simulink model "H175_V3_walk"  (R2025b)
(part 3 of 13)

  L_little1/LConn1 -- L_wrist_yaw1/RConn4
  L_middle1/LConn1 -- L_wrist_yaw1/RConn3
  L_elbow/RConn1 -- L_elbow1/LConn1
  L_ring1/LConn1 -- L_wrist_yaw1/RConn2
  L_thumb1/LConn1 -- L_wrist_yaw1/RConn1
  R_ankle_pitch/RConn1 -- R_ankle_pitch1/LConn1
  R_ankle_pitch1/RConn1 -- R_ankle_roll/LConn1
  R_ankle_roll/RConn1 -- ct_rot_R1/LConn1 -- ct_rot_R2/LConn1 -- ct_rot_R3/LConn1 -- R_ankle_roll1/LConn1 -- ct_rot_R4/LConn1
  R_ankle_roll1/RConn1 -- R_toe/LConn1
  R_clavicle/RConn1 -- R_clavicle1/LConn1
  R_clavicle1/RConn1 -- R_shoulder_pitch/LConn1
  R_elbow/RConn1 -- R_elbow1/LConn1
  R_elbow1/RConn1 -- R_forearm_twist/LConn1
  L_elbow1/RConn1 -- L_forearm_twist/LConn1
  R_forearm_twist/RConn1 -- R_forearm_twist1/LConn1
  R_forearm_twist1/RConn1 -- R_wrist_pitch/LConn1
  R_hip_pitch/RConn1 -- R_hip_pitch1/LConn1
  R_hip_pitch1/RConn1 -- R_hip_roll/LConn1
  R_hip_roll/RConn1 -- R_hip_roll1/LConn1
  R_hip_roll1/RConn1 -- R_hip_yaw/LConn1
  R_hip_yaw/RConn1 -- R_hip_yaw1/LConn1
  R_hip_yaw1/RConn1 -- R_knee/LConn1
  R_index1/RConn1 -- R_index4/LConn1
  R_index2/LConn1 -- R_index4/RConn1
  L_forearm_twist/RConn1 -- L_forearm_twist1/LConn1
  R_index2/RConn1 -- R_index5/LConn1
  R_index3/LConn1 -- R_index5/RConn1
  R_index3/RConn1 -- R_index6/LConn1
  R_knee/RConn1 -- R_knee1/LConn1
  R_ankle_pitch/LConn1 -- R_knee1/RConn1
  R_little1/RConn1 -- R_little4/LConn1
  R_little2/LConn1 -- R_little4/RConn1
  R_little2/RConn1 -- R_little5/LConn1
  R_little3/LConn1 -- R_little5/RConn1
  R_little3/RConn1 -- R_little6/LConn1
  L_forearm_twist1/RConn1 -- L_wrist_pitch/LConn1
  R_middle1/RConn1 -- R_middle4/LConn1
  R_middle2/LConn1 -- R_middle4/RConn1
  R_middle2/RConn1 -- R_middle5/LConn1
  R_middle3/LConn1 -- R_middle5/RConn1
  R_middle3/RConn1 -- R_middle6/LConn1
  R_ring1/RConn1 -- R_ring4/LConn1
  R_ring2/LConn1 -- R_ring4/RConn1
  R_ring2/RConn1 -- R_ring5/LConn1
  R_ring3/LConn1 -- R_ring5/RConn1
  R_ring3/RConn1 -- R_ring6/LConn1
  Solver Configuration/RConn1 -- MechanismConfiguration/RConn1 -- FloatingBase/LConn1 -- GroundTf/LConn1 -- ps_X/LConn1 -- ps_Y/LConn1 -- ps_XDot/LConn1 -- World/RConn1 -- ps_YDot/LConn1
  FloatingBase/RConn1 -- ps_X/RConn1 -- ps_Y/RConn1 -- ps_XDot/RConn1 -- pelvis/LConn1 -- ps_YDot/RConn1
  Ground/RConn1 -- GroundTf/RConn1 -- gnd_L1/RConn1 -- gnd_L2/RConn1 -- gnd_L3/RConn1 -- gnd_L4/RConn1 -- gnd_R1/RConn1 -- gnd_R2/RConn1 -- gnd_R3/RConn1 -- gnd_R4/RConn1
  ct_rot_L1/RConn1 -- ct_tf_L1/LConn1
  ct_tf_L1/RConn1 -- ct_sph_L1/RConn1
  gnd_L1/LConn1 -- Contact_L1/LConn1
  ct_sph_L1/LConn1 -- Contact_L1/RConn1
  ct_rot_L2/RConn1 -- ct_tf_L2/LConn1
  ct_tf_L2/RConn1 -- ct_sph_L2/RConn1
  gnd_L2/LConn1 -- Contact_L2/LConn1
  ct_sph_L2/LConn1 -- Contact_L2/RConn1
  ct_rot_L3/RConn1 -- ct_tf_L3/LConn1
  ct_tf_L3/RConn1 -- ct_sph_L3/RConn1
  gnd_L3/LConn1 -- Contact_L3/LConn1
  ct_sph_L3/LConn1 -- Contact_L3/RConn1
  ct_rot_L4/RConn1 -- ct_tf_L4/LConn1
  ct_tf_L4/RConn1 -- ct_sph_L4/RConn1
  gnd_L4/LConn1 -- Contact_L4/LConn1
  ct_sph_L4/LConn1 -- Contact_L4/RConn1
  ct_rot_R1/RConn1 -- ct_tf_R1/LConn1
  ct_tf_R1/RConn1 -- ct_sph_R1/RConn1
  gnd_R1/LConn1 -- Contact_R1/LConn1
  ct_sph_R1/LConn1 -- Contact_R1/RConn1
  ct_rot_R2/RConn1 -- ct_tf_R2/LConn1
  ct_tf_R2/RConn1 -- ct_sph_R2/RConn1
  gnd_R2/LConn1 -- Contact_R2/LConn1
  ct_sph_R2/LConn1 -- Contact_R2/RConn1
  ct_rot_R3/RConn1 -- ct_tf_R3/LConn1
  ct_tf_R3/RConn1 -- ct_sph_R3/RConn1
  gnd_R3/LConn1 -- Contact_R3/LConn1
  ct_sph_R3/LConn1 -- Contact_R3/RConn1
  ct_rot_R4/RConn1 -- ct_tf_R4/LConn1
  ct_tf_R4/RConn1 -- ct_sph_R4/RConn1
  gnd_R4/LConn1 -- Contact_R4/LConn1
  ct_sph_R4/LConn1 -- Contact_R4/RConn1
  L_ankle_pitch/RConn2 -- cq_L_ankle_pitch/LConn1
  L_ankle_pitch/RConn3 -- cw_L_ankle_pitch/LConn1
  ct_L_ankle_pitch/RConn1 -- L_ankle_pitch/LConn2
  L_ankle_roll/RConn2 -- cq_L_ankle_roll/LConn1
  L_ankle_roll/RConn3 -- cw_L_ankle_roll/LConn1
  ct_L_ankle_roll/RConn1 -- L_ankle_roll/LConn2
  L_clavicle/RConn2 -- cq_L_clavicle/LConn1
  L_clavicle/RConn3 -- cw_L_clavicle/LConn1
  ct_L_clavicle/RConn1 -- L_clavicle/LConn2
  L_elbow/RConn2 -- cq_L_elbow/LConn1
  L_elbow/RConn3 -- cw_L_elbow/LConn1
  ct_L_elbow/RConn1 -- L_elbow/LConn2
  L_forearm_twist/RConn2 -- cq_L_forearm_twist/LConn1
  L_forearm_twist/RConn3 -- cw_L_forearm_twist/LConn1
  ct_L_forearm_twist/RConn1 -- L_forearm_twist/LConn2
  L_hip_pitch/RConn2 -- cq_L_hip_pitch/LConn1
  L_hip_pitch/RConn3 -- cw_L_hip_pitch/LConn1
  ct_L_hip_pitch/RConn1 -- L_hip_pitch/LConn2
  L_hip_roll/RConn2 -- cq_L_hip_roll/LConn1
  L_hip_roll/RConn3 -- cw_L_hip_roll/LConn1
  ct_L_hip_roll/RConn1 -- L_hip_roll/LConn2
  L_hip_yaw/RConn2 -- cq_L_hip_yaw/LConn1
  L_hip_yaw/RConn3 -- cw_L_hip_yaw/LConn1
  ct_L_hip_yaw/RConn1 -- L_hip_yaw/LConn2
  L_index1/RConn2 -- cq_L_index1/LConn1
  L_index1/RConn3 -- cw_L_index1/LConn1
  ct_L_index1/RConn1 -- L_index1/LConn2
  L_index2/RConn2 -- cq_L_index2/LConn1
  L_index2/RConn3 -- cw_L_index2/LConn1
  ct_L_index2/RConn1 -- L_index2/LConn2
  L_index3/RConn2 -- cq_L_index3/LConn1
  L_index3/RConn3 -- cw_L_index3/LConn1
  ct_L_index3/RConn1 -- L_index3/LConn2
  L_knee/RConn2 -- cq_L_knee/LConn1
  L_knee/RConn3 -- cw_L_knee/LConn1
  ct_L_knee/RConn1 -- L_knee/LConn2
  L_little1/RConn2 -- cq_L_little1/LConn1
  L_little1/RConn3 -- cw_L_little1/LConn1
  ct_L_little1/RConn1 -- L_little1/LConn2
  L_little2/RConn2 -- cq_L_little2/LConn1
  L_little2/RConn3 -- cw_L_little2/LConn1
  ct_L_little2/RConn1 -- L_little2/LConn2
  L_little3/RConn2 -- cq_L_little3/LConn1
  L_little3/RConn3 -- cw_L_little3/LConn1
  ct_L_little3/RConn1 -- L_little3/LConn2
  L_middle1/RConn2 -- cq_L_middle1/LConn1
  L_middle1/RConn3 -- cw_L_middle1/LConn1
  ct_L_middle1/RConn1 -- L_middle1/LConn2
  L_middle2/RConn2 -- cq_L_middle2/LConn1
  L_middle2/RConn3 -- cw_L_middle2/LConn1
  ct_L_middle2/RConn1 -- L_middle2/LConn2
  L_middle3/RConn2 -- cq_L_middle3/LConn1
  L_middle3/RConn3 -- cw_L_middle3/LConn1
  ct_L_middle3/RConn1 -- L_middle3/LConn2
  L_ring1/RConn2 -- cq_L_ring1/LConn1
  L_ring1/RConn3 -- cw_L_ring1/LConn1
  ct_L_ring1/RConn1 -- L_ring1/LConn2
  L_ring2/RConn2 -- cq_L_ring2/LConn1
  L_ring2/RConn3 -- cw_L_ring2/LConn1
  ct_L_ring2/RConn1 -- L_ring2/LConn2
  L_ring3/RConn2 -- cq_L_ring3/LConn1
  L_ring3/RConn3 -- cw_L_ring3/LConn1
  ct_L_ring3/RConn1 -- L_ring3/LConn2
  L_scapula/RConn2 -- cq_L_scapula/LConn1
  L_scapula/RConn3 -- cw_L_scapula/LConn1
  ct_L_scapula/RConn1 -- L_scapula/LConn2
  L_shoulder_pitch/RConn2 -- cq_L_shoulder_pitch/LConn1
  L_shoulder_pitch/RConn3 -- cw_L_shoulder_pitch/LConn1
  ct_L_shoulder_pitch/RConn1 -- L_shoulder_pitch/LConn2
  L_shoulder_roll/RConn2 -- cq_L_shoulder_roll/LConn1
  L_shoulder_roll/RConn3 -- cw_L_shoulder_roll/LConn1
  ct_L_shoulder_roll/RConn1 -- L_shoulder_roll/LConn2
  L_shoulder_yaw/RConn2 -- cq_L_shoulder_yaw/LConn1
  L_shoulder_yaw/RConn3 -- cw_L_shoulder_yaw/LConn1
  ct_L_shoulder_yaw/RConn1 -- L_shoulder_yaw/LConn2
  L_thumb1/RConn2 -- cq_L_thumb1/LConn1
  L_thumb1/RConn3 -- cw_L_thumb1/LConn1
  ct_L_thumb1/RConn1 -- L_thumb1/LConn2
  L_thumb2/RConn2 -- cq_L_thumb2/LConn1
  L_thumb2/RConn3 -- cw_L_thumb2/LConn1
  ct_L_thumb2/RConn1 -- L_thumb2/LConn2
  L_thumb3/RConn2 -- cq_L_thumb3/LConn1
  L_thumb3/RConn3 -- cw_L_thumb3/LConn1
  ct_L_thumb3/RConn1 -- L_thumb3/LConn2
  L_toe/RConn2 -- cq_L_toe/LConn1
  L_toe/RConn3 -- cw_L_toe/LConn1
  ct_L_toe/RConn1 -- L_toe/LConn2
  L_wrist_pitch/RConn2 -- cq_L_wrist_pitch/LConn1
  L_wrist_pitch/RConn3 -- cw_L_wrist_pitch/LConn1
  ct_L_wrist_pitch/RConn1 -- L_wrist_pitch/LConn2
  L_wrist_roll/RConn2 -- cq_L_wrist_roll/LConn1
  L_wrist_roll/RConn3 -- cw_L_wrist_roll/LConn1
  ct_L_wrist_roll/RConn1 -- L_wrist_roll/LConn2
  L_wrist_yaw/RConn2 -- cq_L_wrist_yaw/LConn1
  L_wrist_yaw/RConn3 -- cw_L_wrist_yaw/LConn1
  ct_L_wrist_yaw/RConn1 -- L_wrist_yaw/LConn2
  R_ankle_pitch/RConn2 -- cq_R_ankle_pitch/LConn1
  R_ankle_pitch/RConn3 -- cw_R_ankle_pitch/LConn1
  ct_R_ankle_pitch/RConn1 -- R_ankle_pitch/LConn2
  R_ankle_roll/RConn2 -- cq_R_ankle_roll/LConn1
  R_ankle_roll/RConn3 -- cw_R_ankle_roll/LConn1
  ct_R_ankle_roll/RConn1 -- R_ankle_roll/LConn2
  R_clavicle/RConn2 -- cq_R_clavicle/LConn1
  R_clavicle/RConn3 -- cw_R_clavicle/LConn1
  ct_R_clavicle/RConn1 -- R_clavicle/LConn2
  R_elbow/RConn2 -- cq_R_elbow/LConn1
  R_elbow/RConn3 -- cw_R_elbow/LConn1
  ct_R_elbow/RConn1 -- R_elbow/LConn2
  R_forearm_twist/RConn2 -- cq_R_forearm_twist/LConn1
  R_forearm_twist/RConn3 -- cw_R_forearm_twist/LConn1
  ct_R_forearm_twist/RConn1 -- R_forearm_twist/LConn2
  R_hip_pitch/RConn2 -- cq_R_hip_pitch/LConn1
  R_hip_pitch/RConn3 -- cw_R_hip_pitch/LConn1
  ct_R_hip_pitch/RConn1 -- R_hip_pitch/LConn2
  R_hip_roll/RConn2 -- cq_R_hip_roll/LConn1
  R_hip_roll/RConn3 -- cw_R_hip_roll/LConn1
  ct_R_hip_roll/RConn1 -- R_hip_roll/LConn2
  R_hip_yaw/RConn2 -- cq_R_hip_yaw/LConn1
  R_hip_yaw/RConn3 -- cw_R_hip_yaw/LConn1
  ct_R_hip_yaw/RConn1 -- R_hip_yaw/LConn2
  R_index1/RConn2 -- cq_R_index1/LConn1
  R_index1/RConn3 -- cw_R_index1/LConn1
  ct_R_index1/RConn1 -- R_index1/LConn2
  R_index2/RConn2 -- cq_R_index2/LConn1
  R_index2/RConn3 -- cw_R_index2/LConn1
  ct_R_index2/RConn1 -- R_index2/LConn2
  R_index3/RConn2 -- cq_R_index3/LConn1
  R_index3/RConn3 -- cw_R_index3/LConn1
  ct_R_index3/RConn1 -- R_index3/LConn2
  R_knee/RConn2 -- cq_R_knee/LConn1
  R_knee/RConn3 -- cw_R_knee/LConn1
  ct_R_knee/RConn1 -- R_knee/LConn2
  R_little1/RConn2 -- cq_R_little1/LConn1
  R_little1/RConn3 -- cw_R_little1/LConn1
  ct_R_little1/RConn1 -- R_little1/LConn2
  R_little2/RConn2 -- cq_R_little2/LConn1
  R_little2/RConn3 -- cw_R_little2/LConn1
  ct_R_little2/RConn1 -- R_little2/LConn2
  R_little3/RConn2 -- cq_R_little3/LConn1
  R_little3/RConn3 -- cw_R_little3/LConn1
  ct_R_little3/RConn1 -- R_little3/LConn2
  R_middle1/RConn2 -- cq_R_middle1/LConn1
  R_middle1/RConn3 -- cw_R_middle1/LConn1
  ct_R_middle1/RConn1 -- R_middle1/LConn2
  R_middle2/RConn2 -- cq_R_middle2/LConn1
  R_middle2/RConn3 -- cw_R_middle2/LConn1
  ct_R_middle2/RConn1 -- R_middle2/LConn2
  R_middle3/RConn2 -- cq_R_middle3/LConn1
  R_middle3/RConn3 -- cw_R_middle3/LConn1
  ct_R_middle3/RConn1 -- R_middle3/LConn2
  R_ring1/RConn2 -- cq_R_ring1/LConn1
  R_ring1/RConn3 -- cw_R_ring1/LConn1
  ct_R_ring1/RConn1 -- R_ring1/LConn2
  R_ring2/RConn2 -- cq_R_ring2/LConn1
  R_ring2/RConn3 -- cw_R_ring2/LConn1
  ct_R_ring2/RConn1 -- R_ring2/LConn2
  R_ring3/RConn2 -- cq_R_ring3/LConn1
  R_ring3/RConn3 -- cw_R_ring3/LConn1
  ct_R_ring3/RConn1 -- R_ring3/LConn2
  R_scapula/RConn2 -- cq_R_scapula/LConn1
  R_scapula/RConn3 -- cw_R_scapula/LConn1
  ct_R_scapula/RConn1 -- R_scapula/LConn2
  R_shoulder_pitch/RConn2 -- cq_R_shoulder_pitch/LConn1
  R_shoulder_pitch/RConn3 -- cw_R_shoulder_pitch/LConn1
  ct_R_shoulder_pitch/RConn1 -- R_shoulder_pitch/LConn2
  R_shoulder_roll/RConn2 -- cq_R_shoulder_roll/LConn1
  R_shoulder_roll/RConn3 -- cw_R_shoulder_roll/LConn1
  ct_R_shoulder_roll/RConn1 -- R_shoulder_roll/LConn2
  R_shoulder_yaw/RConn2 -- cq_R_shoulder_yaw/LConn1
  R_shoulder_yaw/RConn3 -- cw_R_shoulder_yaw/LConn1
  ct_R_shoulder_yaw/RConn1 -- R_shoulder_yaw/LConn2
  R_thumb1/RConn2 -- cq_R_thumb1/LConn1
  R_thumb1/RConn3 -- cw_R_thumb1/LConn1
  ct_R_thumb1/RConn1 -- R_thumb1/LConn2
  R_thumb2/RConn2 -- cq_R_thumb2/LConn1
  R_thumb2/RConn3 -- cw_R_thumb2/LConn1
  ct_R_thumb2/RConn1 -- R_thumb2/LConn2
  R_thumb3/RConn2 -- cq_R_thumb3/LConn1
  R_thumb3/RConn3 -- cw_R_thumb3/LConn1
  ct_R_thumb3/RConn1 -- R_thumb3/LConn2
  R_toe/RConn2 -- cq_R_toe/LConn1
  R_toe/RConn3 -- cw_R_toe/LConn1
  ct_R_toe/RConn1 -- R_toe/LConn2
  R_wrist_pitch/RConn2 -- cq_R_wrist_pitch/LConn1
  R_wrist_pitch/RConn3 -- cw_R_wrist_pitch/LConn1
  ct_R_wrist_pitch/RConn1 -- R_wrist_pitch/LConn2
  R_wrist_roll/RConn2 -- cq_R_wrist_roll/LConn1
  R_wrist_roll/RConn3 -- cw_R_wrist_roll/LConn1
  ct_R_wrist_roll/RConn1 -- R_wrist_roll/LConn2
  R_wrist_yaw/RConn2 -- cq_R_wrist_yaw/LConn1
  R_wrist_yaw/RConn3 -- cw_R_wrist_yaw/LConn1
  ct_R_wrist_yaw/RConn1 -- R_wrist_yaw/LConn2
  neck_pitch/RConn2 -- cq_neck_pitch/LConn1
  neck_pitch/RConn3 -- cw_neck_pitch/LConn1
  ct_neck_pitch/RConn1 -- neck_pitch/LConn2
  neck_roll/RConn2 -- cq_neck_roll/LConn1
  neck_roll/RConn3 -- cw_neck_roll/LConn1
  ct_neck_roll/RConn1 -- neck_roll/LConn2
  neck_yaw/RConn2 -- cq_neck_yaw/LConn1
  neck_yaw/RConn3 -- cw_neck_yaw/LConn1
  ct_neck_yaw/RConn1 -- neck_yaw/LConn2
  waist_pitch/RConn2 -- cq_waist_pitch/LConn1
  waist_pitch/RConn3 -- cw_waist_pitch/LConn1
  ct_waist_pitch/RConn1 -- waist_pitch/LConn2
  waist_roll/RConn2 -- cq_waist_roll/LConn1
  waist_roll/RConn3 -- cw_waist_roll/LConn1
  ct_waist_roll/RConn1 -- waist_roll/LConn2
  waist_yaw/RConn2 -- cq_waist_yaw/LConn1
  waist_yaw/RConn3 -- cw_waist_yaw/LConn1
  ct_waist_yaw/RConn1 -- waist_yaw/LConn2
  ps_X/RConn2 -- pc_X/LConn1
  ps_Y/RConn2 -- pc_Y/LConn1
  ps_XDot/RConn2 -- pc_XDot/LConn1
  ps_YDot/RConn2 -- pc_YDot/LConn1
